simulink model "EINT_RL_closed_loop_yaw"  (R2025a)
settings: Solver=FixedStepAuto  StartTime=0.0  StopTime=T_end  FixedStep=Ts  RelTol=1e-3
values from neighbouring files (symbols this model uses):
  Ts = 0.05    [EINT_RL_eval_yaw.m]    (also in rl_controller_full.m)
settings Model: Creator=LOQ  LastModifiedBy=LOQ

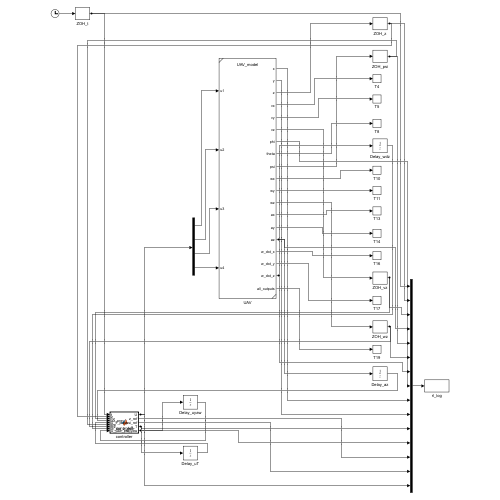
[thumbnail: Simulink's stored preview of the top-level diagram]
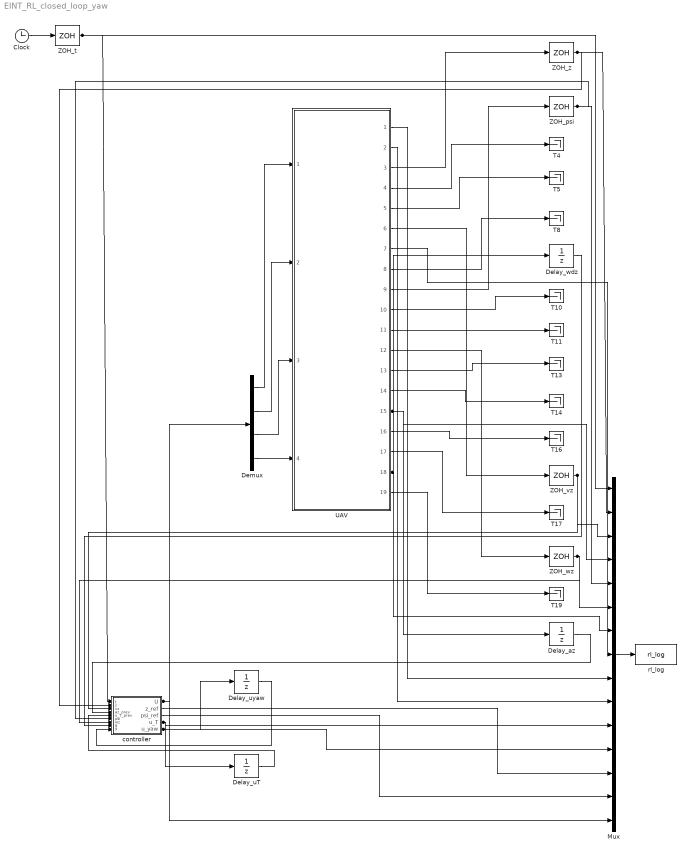
== system EINT_RL_closed_loop_yaw ==
  Clock : Clock
  Delay_az : UnitDelay  SampleTime=Ts  HasFrameUpgradeWarning=on
  Delay_uT : UnitDelay  SampleTime=Ts  HasFrameUpgradeWarning=on
  Delay_uyaw : UnitDelay  SampleTime=Ts  HasFrameUpgradeWarning=on
  Delay_wdz : UnitDelay  SampleTime=Ts  HasFrameUpgradeWarning=on
  Demux : Demux
  Mux : Mux  Inputs=15
  T{4..5,8,10..11,13..14,16..17,19} (10 alike) : Terminator
  UAV : Subsystem  ReferencedSubsystem=UAV_model
  ZOH_psi : ZeroOrderHold  SampleTime=Ts
  ZOH_t : ZeroOrderHold  SampleTime=Ts
  ZOH_vz : ZeroOrderHold  SampleTime=Ts
  ZOH_wz : ZeroOrderHold  SampleTime=Ts
  ZOH_z : ZeroOrderHold  SampleTime=Ts
  controller : MATLAB Function  TreatAsAtomicUnit=on
  rl_log : ToWorkspace  VariableName=rl_log  SampleTime=Ts
  wires:
  Clock/1 -> ZOH_t/1
  controller/5(u_yaw) -> Delay_uyaw/1, Mux/12
  controller/3(psi_ref) -> Mux/14
  ZOH_t/1 -> Mux/1, controller/1(t)
  controller/4(u_T) -> Mux/11, Delay_uT/1
  ZOH_vz/1 -> controller/3(vz), Mux/3
  controller/2(z_ref) -> Mux/13
  controller/1(U) -> Mux/15, Demux/1
  Delay_az/1 -> controller/4(az_prev)
  Demux/1 -> UAV/1
  Demux/2 -> UAV/2
  Demux/3 -> UAV/3
  Delay_wdz/1 -> controller/8(w_dot_z_prev)
  Demux/4 -> UAV/4
  Delay_uyaw/1 -> controller/9(u_yaw_prev)
  Delay_uT/1 -> controller/5(u_T_prev)
  UAV/17 -> T17/1
  UAV/1 -> Mux/9
  UAV/18 -> Mux/7, Delay_wdz/1
  UAV/2 -> Mux/10
  UAV/19 -> T19/1
  UAV/3 -> ZOH_z/1
  UAV/4 -> T4/1
  UAV/5 -> T5/1
  UAV/6 -> ZOH_vz/1
  UAV/7 -> Mux/8
  UAV/8 -> T8/1
  UAV/9 -> ZOH_psi/1
  UAV/10 -> T10/1
  UAV/11 -> T11/1
  UAV/12 -> ZOH_wz/1
  UAV/13 -> T13/1
  UAV/14 -> T14/1
  UAV/15 -> Mux/4, Delay_az/1
  UAV/16 -> T16/1
  ZOH_z/1 -> Mux/2, controller/2(z)
  ZOH_psi/1 -> controller/6(psi), Mux/5
  ZOH_wz/1 -> controller/7(wz), Mux/6
  Mux/1 -> rl_log/1

== matlab function EINT_RL_closed_loop_yaw/controller ==
  data: t input; U output; z input; vz input; az_prev input; u_T_prev input; psi input; wz input; w_dot_z_prev input; u_yaw_prev input; z_ref output; psi_ref output; u_T output; u_yaw output
function [U, z_ref, psi_ref, u_T, u_yaw] = controller(t, z, vz, az_prev, u_T_prev, psi, wz, w_dot_z_prev, u_yaw_prev)
coder.extrinsic('rl_controller_full');
U = zeros(4, 1); z_ref = 0; psi_ref = 0; u_T = 0; u_yaw = 0;
[U, z_ref, psi_ref, u_T, u_yaw] = rl_controller_full(t, z, vz, az_prev, u_T_prev, psi, wz, w_dot_z_prev, u_yaw_prev);
